simulink model "ASM_Traffic_MultiCore"  (R2026a)
settings: Solver=ode1  StartTime=SIM.tstart.v  StopTime=SIM.tend.v  FixedStep=SIM.StepSize.v
PostLoadFcn:
  | if any(exist('dsrtsu_mdlpostloadfcn', 'file') ~= 0), dsrtsu_mdlpostloadfcn('Execute', bdroot); end
  | try, asm_mdl_postloadfcn(bdroot, 'UpdateModel', 3600); catch, disp(lasterr); end,
InitFcn:
  | , if any(exist('rtifpga_mdlclblib', 'file') ~= 0), rtifpga_mdlclblib('Init', bdroot); end,
  | , if any(exist('dsmpb_private', 'file') ~= 0), dsmpb_private('dsmpb_mdlclblib', 'Init', bdroot); end,
model workspace (MAT data in the model file):
  asmReferencePath = [0 0.01 0.02 0.03 0.04 0.05 0.06 0.07 0.08 0.09 0.1 0.11 ... (350007 elements, 50001x7)]
  roadBounds : Simulink.Parameter (value not decoded)
  safetyAxes : Simulink.Parameter (value not decoded)
undefined symbols (not defined in the file): _to_, a0b2, ASM_BrakeHydraulics_DemoSystems, ASM_VehicleDynamics_DemoSystems, b98103fe8ad365046cd0, BrakeCircuit, controllerConfig, CPT, Crankshaft, DiscIntNeverNeededParam, dsmsi, FinalDriveAssembly, MDL, ModeSignals, mu, Pos_BrakePedal_Maneuver, rad, RefSignals, roadFamilyData, roadFamilyId, s_to_rpm, SIM, SoftECU, Suspension, Tire, Transmission
libraries: ASM_Traffic_lib x135, simulink x98, ASM_Utils_lib x77, ASM_VehicleDynamics_lib x70, ASM_Environment_lib x22, dsmpblib x20, dsmsilib x15, MDLD_Utils_lib x10, ASM_BrakeHydraulics_lib x3, sl_discontinuities x2
(part 7 of 65)

== system ASM_Traffic_MultiCore/AnimationInterface/ANIMATION_INTERFACE/ASM_Vehicle_Instruments ==
  VehicleDynamics_Animation : Inport
  Environment_Animation : Inport  Port=2
  Drivetrain_Animation : Inport  Port=3
  Bus Selector1 : BusSelector  OutputSignals=v_x_Vehicle_CoG[km|h],a_y_Vehicle_CoG[m|s2],YawRate_Vehicle_CoG[deg|s]
  Bus Selector15 : BusSelector  OutputSignals=n_Engine[rpm],Gear[]
  Bus Selector2 : BusSelector  OutputSignals=s_Vehicle[m],Angle_Yaw_Vehicle_CoorSys_E[deg]
  Bus Selector4 : BusSelector  OutputSignals=s_Veh_Road[m],ManeuverTime[s],ManeuverState[]
  Enable_Data_Transfer : Constant
  Vehicle_Instruments : dsmsilib/dsmsi_simulation_data_objects_BL1  Priority=10001  parameterStr="{\"Version\":1,\"TransformInput\":false,\"EnableInput\":true,\"Objects\":[{\"Oid\":1,\"Name\":\"Speed\",\"TypeClass\":{\"Name\":\"Signal\",\"Class\":3,\"SignalProperty\":{\"InstrumentInput\":\"Input port\",\"Description\":null,\"Unit\":\"km/h\",\"Type\":0,\"Length\":1,\"ObjectsCount\":1},\"TransformationProperty\":null,\"PositionAndScaleProperty\":null,\"PositionProperty\":null},\"Children\":[]},{\"Oid\":2,\"Name\":\"LatAcc\",\"TypeClass\":{\"Name\":\"Signal\",\"Class\":3,\"SignalProperty\":{\"InstrumentInput\":\"Input port\",\"Description\":null,\"Unit\":\"m/s2\",\"Type\":0,\"Length\":1,\"ObjectsCount\":1},\"TransformationProperty\":null,\"PositionAndScaleProperty\":null,\"PositionProperty\":null},\"Children\":[]},{\"Oid\":3,\"Name\":\"YawRate\",\"TypeClass\":{\"Name\":\"Signal\",\"Class\":3,\"SignalProperty\":{\"InstrumentInput\":\"Input port\",\"Description\":null,\"Unit\":\"deg/s\",\"Type\":0,\"Length\":1,\"ObjectsCount\":1},\"TransformationProperty\":null,\"PositionAndScaleProperty\":null,\"PositionProperty\":null},\"Children\":[]},{\"Oid\":4,\"Name\":\"Engine\",\"TypeClass\":{\"Name\":\"Signal\",\"Class\":3,\"SignalProperty\":{\"InstrumentInput\":\"Input port\",\"Description\":null,\"Unit\":\"rpm\",\"Type\":0,\"Length\":1,\"ObjectsCount\":1},\"TransformationProperty\":null,\"PositionAndScaleProperty\":null,\"PositionProperty\":null},\"Children\":[]},{\"Oid\":5,\"Name\":\"Gear\",\"TypeClass\":{\"Name\":\"Signal\",\"Class\":3,\"SignalProperty\":{\"InstrumentInput\":\"Input port\",\"Description\":null,\"Unit\":null,\"Type\":0,\"Length\":1,\"ObjectsCount\":1},\"TransformationProperty\":null,\"PositionAndScaleProperty\":null,\"PositionProperty\":null},\"Children\":[]},{\"Oid\":6,\"Name\":\"s_Road\",\"TypeClass\":{\"Name\":\"Signal\",\"Class\":3,\"SignalProperty\":{\"InstrumentInput\":\"Input port\",\"Description\":null,\"Unit\":\"m\",\"Type\":0,\"Length\":1,\"ObjectsCount\":1},\"TransformationProperty\":null,\"PositionAndScaleProperty\":null,\"PositionProperty\":null},\"Children\":[]},{\"Oid\":7,\"Name\":\"ManeuverTime\",\"TypeClass\":{\"Name\":\"Signal\",\"Class\":3,\"SignalProperty\":{\"InstrumentInput\":\"Input port\",\"Description\":null,\"Unit\":\"s\",\"Type\":0,\"Length\":1,\"ObjectsCount\":1},\"TransformationProperty\":null,\"PositionAndScaleProperty\":null,\"PositionProperty\":null},\"Children\":[]},{\"Oid\":8,\"Name\":\"ManeuverState\",\"TypeClass\":{\"Name\":\"Signal\",\"Class\":3,\"SignalProperty\":{\"InstrumentInput\":\"Input port\",\"Description\":null,\"Unit\":null,\"Type\":0,\"Length\":1,\"ObjectsCount\":1},\"TransformationProperty\":null,\"PositionAndScaleProperty\":null,\"PositionProperty\":null},\"Children\":[]},{\"Oid\":9,\"Name\":\"DrivenDistance\",\"TypeClass\":{\"Name\":\"Signal\",\"Class\":3,\"SignalProperty\":{\"InstrumentInput\":\"Input port\",\"Description\":null,\"Unit\":\"m\",\"Type\":0,\"Length\":1,\"ObjectsCount\":1},\"TransformationProperty\":null,\"PositionAndScaleProperty\":null,\"PositionProperty\":null},\"Children\":[]},{\"Oid\":10,\"Name\":\"YawAngle\",\"TypeClass\":{\"Name\":\"Signal\",\"Class\":3,\"SignalProperty\":{\"InstrumentInput\":\"Input port\",\"Description\":null,\"Unit\":\"deg\",\"Type\":0,\"Length\":1,\"ObjectsCount\":1},\"TransformationProperty\":null,\"PositionAndScaleProperty\":null,\"PositionProperty\":null},\"Children\":[]}]}"  evalStr=dsmsi(gcb, 'EvalJson')  sampleTime=-1  globalBlockId=0  objectsBlockId=dsmsi(gcb, 'GetObjectBlockId')  objectsBlockGuiOpen=dsmsi(gcb, 'GetSdoGuiStatus')  dialogIsOpen=0  blockVersion=60  highPrecision=0  validNameBckp=Vehicle_Instruments
      settings: SourceProductName=dSPACE MSI Blockset
  wires:
  Enable_Data_Transfer/1 -> Vehicle_Instruments/1
  Environment_Animation/1 -> Bus Selector4/1
  Bus Selector2/2 -> Vehicle_Instruments/11  "<Angle_Yaw_Vehicle_CoorSys_E[deg]>"
  Bus Selector2/1 -> Vehicle_Instruments/10  "<s_Vehicle[m]>"
  Bus Selector4/1 -> Vehicle_Instruments/7  "<s_Veh_Road[m]>"
  Bus Selector4/2 -> Vehicle_Instruments/8  "<ManeuverTime[s]>"
  Bus Selector1/2 -> Vehicle_Instruments/3  "<a_y_Vehicle_CoG[m|s2]>"
  Bus Selector1/1 -> Vehicle_Instruments/2  "<v_x_Vehicle_CoG[km|h]>"
  Bus Selector1/3 -> Vehicle_Instruments/4  "<YawRate_Vehicle_CoG[deg|s]>"
  Bus Selector4/3 -> Vehicle_Instruments/9  "<ManeuverState[]>"
  VehicleDynamics_Animation/1 -> Bus Selector1/1, Bus Selector2/1
  Drivetrain_Animation/1 -> Bus Selector15/1
  Bus Selector15/1 -> Vehicle_Instruments/5  "<n_Engine[rpm]>"
  Bus Selector15/2 -> Vehicle_Instruments/6  "<Gear[]>"

== system ASM_Traffic_MultiCore/AnimationInterface/ANIMATION_INTERFACE/ASM_Vehicle_Occupants ==
  Environment_Animation : Inport
  Bus Selector : BusSelector  OutputSignals=UserSignals_Customized.DriverMonitoring.DriverGazeLocation[],UserSignals_Customized.DriverMonitoring.DriverAnimation[],UserSignals_Customized.DriverMonitoring.DriverLizardOwlRatio[]
  Enable_Data_Transfer : Constant
  Vehicle_Occupants : dsmsilib/dsmsi_simulation_data_objects_BL1  Priority=10001  parameterStr="{\"Version\":1,\"TransformInput\":false,\"EnableInput\":true,\"Objects\":[{\"Oid\":1,\"Name\":\"Driver\",\"TypeClass\":{\"Name\":\"Transformation\",\"Class\":1,\"SignalProperty\":null,\"TransformationProperty\":{\"ObjectsCount\":1,\"TransformMatrixIn\":false,\"TransformMatrixOut\":false,\"AngleInterpretation\":0,\"TransformationOrder\":0,\"RotationOrder\":0,\"TranslationAsParameter\":true,\"Translation\":\"[0 0 0]\",\"RotationAsParameter\":true,\"Rotation\":\"[0 0 0]\",\"ScalingAsParameter\":true,\"Scaling\":\"[1 1 1]\"},\"PositionAndScaleProperty\":null,\"PositionProperty\":null},\"Children\":[{\"Oid\":2,\"Name\":\"DMS_GazeLocation\",\"TypeClass\":{\"Name\":\"Signal\",\"Class\":3,\"SignalProperty\":{\"ObjectsCount\":1,\"InstrumentInput\":\"Input port\",\"Description\":null,\"Unit\":null,\"Type\":0,\"Length\":1},\"TransformationProperty\":null,\"PositionAndScaleProperty\":null,\"PositionProperty\":null},\"Children\":[]},{\"Oid\":3,\"Name\":\"DMS_DriverAnimation\",\"TypeClass\":{\"Name\":\"Signal\",\"Class\":3,\"SignalProperty\":{\"ObjectsCount\":1,\"InstrumentInput\":\"Input port\",\"Description\":null,\"Unit\":null,\"Type\":0,\"Length\":1},\"TransformationProperty\":null,\"PositionAndScaleProperty\":null,\"PositionProperty\":null},\"Children\":[]},{\"Oid\":4,\"Name\":\"DMS_LizardOwlRatio\",\"TypeClass\":{\"Name\":\"Signal\",\"Class\":3,\"SignalProperty\":{\"ObjectsCount\":1,\"InstrumentInput\":\"Input port\",\"Description\":null,\"Unit\":null,\"Type\":0,\"Length\":1},\"TransformationProperty\":null,\"PositionAndScaleProperty\":null,\"PositionProperty\":null},\"Children\":[]}]}]}"  evalStr=dsmsi(gcb, 'EvalJson')  sampleTime=-1  globalBlockId=0  objectsBlockId=dsmsi(gcb, 'GetObjectBlockId')  objectsBlockGuiOpen=dsmsi(gcb, 'GetSdoGuiStatus')  dialogIsOpen=0  blockVersion=60  highPrecision=0  validNameBckp=Vehicle_Occupants
      settings: SourceProductName=dSPACE MSI Blockset
  wires:
  Bus Selector/3 -> Vehicle_Occupants/4  "<DriverLizardOwlRatio[]>"
  Bus Selector/2 -> Vehicle_Occupants/3  "<DriverAnimation[]>"
  Bus Selector/1 -> Vehicle_Occupants/2  "<DriverGazeLocation[]>"
  Enable_Data_Transfer/1 -> Vehicle_Occupants/1
  Environment_Animation/1 -> Bus Selector/1

== system ASM_Traffic_MultiCore/AnimationInterface/ANIMATION_INTERFACE/Activate_Animation ==

== system ASM_Traffic_MultiCore/AnimationInterface/ANIMATION_INTERFACE/Activate_Animation1 ==

== system ASM_Traffic_MultiCore/AnimationInterface/ANIMATION_INTERFACE/Activate_Animation2 ==

== system ASM_Traffic_MultiCore/AnimationInterface/ANIMATION_INTERFACE/Activate_Animation3 ==

== system ASM_Traffic_MultiCore/AnimationInterface/ANIMATION_INTERFACE/Activate_Animation4 ==

== system ASM_Traffic_MultiCore/AnimationInterface/ANIMATION_INTERFACE/Activate_Animation5 ==

== system ASM_Traffic_MultiCore/AnimationInterface/ANIMATION_INTERFACE/Activate_Animation6 ==

== system ASM_Traffic_MultiCore/AnimationInterface/ANIMATION_INTERFACE/Bounding_Boxes ==
  Environment_Animation : Inport
  BoundingBox_1 : Subsystem
  BoundingBox_10 : Subsystem
  BoundingBox_2 : Subsystem
  BoundingBox_3 : Subsystem
  BoundingBox_4 : Subsystem
  BoundingBox_5 : Subsystem
  BoundingBox_6 : Subsystem
  BoundingBox_7 : Subsystem
  BoundingBox_8 : Subsystem
  BoundingBox_9 : Subsystem
  Bounding_Boxes : dsmsilib/dsmsi_simulation_data_objects_BL1  Priority=10001  parameterStr="{\"Version\":1,\"TransformInput\":false,\"EnableInput\":true,\"Objects\":[{\"Name\":\"Boundingbox_01\",\"TypeClass\":{\"Name\":\"Transformation\",\"Class\":1,\"SignalProperty\":null,\"TransformationProperty\":{\"TransformMatrixIn\":false,\"TransformMatrixOut\":false,\"AngleInterpretation\":0,\"TransformationOrder\":0,\"RotationOrder\":0,\"TranslationAsParameter\":false,\"Translation\":\"[0 0 0]\",\"RotationAsParameter\":false,\"Rotation\":\"[0 0 0]\",\"ScalingAsParameter\":false,\"Scaling\":\"[1 1 1]\",\"ObjectsCount\":1},\"PositionAndScaleProperty\":null,\"PositionProperty\":null},\"Children\":[],\"Oid\":1},{\"Name\":\"Boundingbox_02\",\"TypeClass\":{\"Name\":\"Transformation\",\"Class\":1,\"SignalProperty\":null,\"TransformationProperty\":{\"TransformMatrixIn\":false,\"TransformMatrixOut\":false,\"AngleInterpretation\":0,\"TransformationOrder\":0,\"RotationOrder\":0,\"TranslationAsParameter\":false,\"Translation\":\"[0 0 0]\",\"RotationAsParameter\":false,\"Rotation\":\"[0 0 0]\",\"ScalingAsParameter\":false,\"Scaling\":\"[1 1 1]\",\"ObjectsCount\":1},\"PositionAndScaleProperty\":null,\"PositionProperty\":null},\"Children\":[],\"Oid\":2},{\"Name\":\"Boundingbox_03\",\"TypeClass\":{\"Name\":\"Transformation\",\"Class\":1,\"SignalProperty\":null,\"TransformationProperty\":{\"TransformMatrixIn\":false,\"TransformMatrixOut\":false,\"AngleInterpretation\":0,\"TransformationOrder\":0,\"RotationOrder\":0,\"TranslationAsParameter\":false,\"Translation\":\"[0 0 0]\",\"RotationAsParameter\":false,\"Rotation\":\"[0 0 0]\",\"ScalingAsParameter\":false,\"Scaling\":\"[1 1 1]\",\"ObjectsCount\":1},\"PositionAndScaleProperty\":null,\"PositionProperty\":null},\"Children\":[],\"Oid\":3},{\"Name\":\"Boundingbox_04\",\"TypeClass\":{\"Name\":\"Transformation\",\"Class\":1,\"SignalProperty\":null,\"TransformationProperty\":{\"TransformMatrixIn\":false,\"TransformMatrixOut\":false,\"AngleInterpretation\":0,\"TransformationOrder\":0,\"RotationOrder\":0,\"TranslationAsParameter\":false,\"Translation\":\"[0 0 0]\",\"RotationAsParameter\":false,\"Rotation\":\"[0 0 0]\",\"ScalingAsParameter\":false,\"Scaling\":\"[1 1 1]\",\"ObjectsCount\":1},\"PositionAndScaleProperty\":null,\"PositionProperty\":null},\"Children\":[],\"Oid\":4},{\"Name\":\"Boundingbox_05\",\"TypeClass\":{\"Name\":\"Transformation\",\"Class\":1,\"SignalProperty\":null,\"TransformationProperty\":{\"TransformMatrixIn\":false,\"TransformMatrixOut\":false,\"AngleInterpretation\":0,\"TransformationOrder\":0,\"RotationOrder\":0,\"TranslationAsParameter\":false,\"Translation\":\"[0 0 0]\",\"RotationAsParameter\":false,\"Rotation\":\"[0 0 0]\",\"ScalingAsParameter\":false,\"Scaling\":\"[1 1 1]\",\"ObjectsCount\":1},\"PositionAndScaleProperty\":null,\"PositionProperty\":null},\"Children\":[],\"Oid\":5},{\"Name\":\"Boundingbox_06\",\"TypeClass\":{\"Name\":\"Transformation\",\"Class\":1,\"SignalProperty\":null,\"TransformationProperty\":{\"TransformMatrixIn\":false,\"TransformMatrixOut\":false,\"AngleInterpretation\":0,\"TransformationOrder\":0,\"RotationOrder\":0,\"TranslationAsParameter\":false,\"Translation\":\"[0 0 0]\",\"RotationAsParameter\":false,\"Rotation\":\"[0 0 0]\",\"ScalingAsParameter\":false,\"Scaling\":\"[1 1 1]\",\"ObjectsCount\":1},\"PositionAndScaleProperty\":null,\"PositionProperty\":null},\"Children\":[],\"Oid\":6},{\"Name\":\"Boundingbox_07\",\"TypeClass\":{\"Name\":\"Transformation\",\"Class\":1,\"SignalProperty\":null,\"TransformationProperty\":{\"TransformMatrixIn\":false,\"TransformMatrixOut\":false,\"AngleInterpretation\":0,\"TransformationOrder\":0,\"RotationOrder\":0,\"TranslationAsParameter\":false,\"Translation\":\"[0 0 0]\",\"RotationAsParameter\":false,\"Rotation\":\"[0 0 0]\",\"ScalingAsParameter\":false,\"Scaling\":\"[1 1 1]\",\"ObjectsCount\":1},\"PositionAndScaleProperty\":null,\"PositionProperty\":null},\"Children\":[],\"Oid\":7},{\"Name\":\"Boundingbox_08\",\"TypeClass\":{\"Name\":\"Transformation\",\"Class\":1,\"SignalProperty\":null,\"TransformationProperty\":{\"TransformMatrixIn\":false,\"TransformMatrixOut\":false,\"AngleInterpretation\":0,\"TransformationOrder\":0,\"RotationOrder\":0,\"TranslationAsParameter\":false,\"Translation\":\"[0 0 0]\",\"RotationAsParameter\":false,\"Rotation\":\"[0 0 0]\",\"ScalingAsParameter\":false,\"Scaling\":\"[1 1 1]\",\"ObjectsCount\":1},\"PositionAndScaleProperty\":null,\"PositionProperty\":null},\"Children\":[],\"Oid\":8},{\"Name\":\"Boundingbox_09\",\"TypeClass\":{\"Name\":\"Transformation\",\"Class\":1,\"SignalProperty\":null,\"TransformationProperty\":{\"TransformMatrixIn\":false,\"TransformMatrixOut\":false,\"AngleInterpretation\":0,\"TransformationOrder\":0,\"RotationOrder\":0,\"TranslationAsParameter\":false,\"Translation\":\"[0 0 0]\",\"RotationAsParameter\":false,\"Rotation\":\"[0 0 0]\",\"ScalingAsParameter\":false,\"Scaling\":\"[1 1 1]\",\"ObjectsCount\":1},\"PositionAndScaleProperty\":null,\"PositionProperty\":null},\"Children\":[],\"Oid\":9},{\"Name\":\"Boundingbox_10\",\"TypeClass\":{\"Name\":\"Transformation\",\"Class\":1,\"SignalProperty\":null,\"TransformationProperty\":{\"TransformMatrixIn\":false,\"TransformMatrixOut\":false,\"AngleInterpretation\":0,\"TransformationOrder\":0,\"RotationOrder\":0,\"TranslationAsParameter\":false,\"Translation\":\"[0 0 0]\",\"RotationAsParameter\":false,\"Rotation\":\"[0 0 0]\",\"ScalingAsParameter\":false,\"Scaling\":\"[1 1 1]\",\"ObjectsCount\":1},\"PositionAndScaleProperty\":null,\"PositionProperty\":null},\"Children\":[],\"Oid\":10}]}"  evalStr=dsmsi(gcb, 'EvalJson')  sampleTime=-1  globalBlockId=0  objectsBlockId=dsmsi(gcb, 'GetObjectBlockId')  objectsBlockGuiOpen=dsmsi(gcb, 'GetSdoGuiStatus')  dialogIsOpen=0  blockVersion=60  highPrecision=0  validNameBckp=Bounding_Boxes
      settings: SourceProductName=dSPACE MSI Blockset
  Constant : Constant
  Constant1 : Constant  Value=2
  Constant2 : Constant  Value=3
  Constant3 : Constant  Value=4
  Constant4 : Constant  Value=5
  Constant5 : Constant  Value=6
  Constant6 : Constant  Value=7
  Constant7 : Constant  Value=8
  Constant8 : Constant  Value=9
  Constant9 : Constant  Value=10
  EnableBoxVisualization : Subsystem
  Enable_Data_Transfer : Constant
  wires:
  Enable_Data_Transfer/1 -> Bounding_Boxes/1
  BoundingBox_9/1(Pos_CoorSysE[m]) -> Bounding_Boxes/26
  BoundingBox_9/2(Angle_CoorSysE[m]) -> Bounding_Boxes/27
  BoundingBox_9/3(Dimensions[m]) -> Bounding_Boxes/28
  BoundingBox_10/1(Pos_CoorSysE[m]) -> Bounding_Boxes/29
  BoundingBox_10/2(Angle_CoorSysE[m]) -> Bounding_Boxes/30
  BoundingBox_10/3(Dimensions[m]) -> Bounding_Boxes/31
  BoundingBox_5/1(Pos_CoorSysE[m]) -> Bounding_Boxes/14
  BoundingBox_5/2(Angle_CoorSysE[m]) -> Bounding_Boxes/15
  BoundingBox_5/3(Dimensions[m]) -> Bounding_Boxes/16
  BoundingBox_6/1(Pos_CoorSysE[m]) -> Bounding_Boxes/17
  BoundingBox_6/2(Angle_CoorSysE[m]) -> Bounding_Boxes/18
  BoundingBox_6/3(Dimensions[m]) -> Bounding_Boxes/19
  BoundingBox_8/3(Dimensions[m]) -> Bounding_Boxes/25
  BoundingBox_8/2(Angle_CoorSysE[m]) -> Bounding_Boxes/24
  BoundingBox_8/1(Pos_CoorSysE[m]) -> Bounding_Boxes/23
  BoundingBox_7/3(Dimensions[m]) -> Bounding_Boxes/22
  BoundingBox_7/2(Angle_CoorSysE[m]) -> Bounding_Boxes/21
  BoundingBox_7/1(Pos_CoorSysE[m]) -> Bounding_Boxes/20
  BoundingBox_3/1(Pos_CoorSysE[m]) -> Bounding_Boxes/8
  BoundingBox_3/2(Angle_CoorSysE[m]) -> Bounding_Boxes/9
  BoundingBox_3/3(Dimensions[m]) -> Bounding_Boxes/10
  BoundingBox_4/1(Pos_CoorSysE[m]) -> Bounding_Boxes/11
  BoundingBox_4/2(Angle_CoorSysE[m]) -> Bounding_Boxes/12
  BoundingBox_4/3(Dimensions[m]) -> Bounding_Boxes/13
  BoundingBox_2/3(Dimensions[m]) -> Bounding_Boxes/7
  BoundingBox_2/2(Angle_CoorSysE[m]) -> Bounding_Boxes/6
  BoundingBox_2/1(Pos_CoorSysE[m]) -> Bounding_Boxes/5
  EnableBoxVisualization/1(BoundigBoxes_Animation) -> BoundingBox_10/2(BoundigBoxes_Animation), BoundingBox_9/2(BoundigBoxes_Animation), BoundingBox_8/2(BoundigBoxes_Animation), BoundingBox_7/2(BoundigBoxes_Animation), BoundingBox_6/2(BoundigBoxes_Animation), BoundingBox_5/2(BoundigBoxes_Animation), BoundingBox_4/2(BoundigBoxes_Animation), BoundingBox_3/2(BoundigBoxes_Animation), BoundingBox_2/2(BoundigBoxes_Animation), BoundingBox_1/2(BoundigBoxes_Animation)
  Environment_Animation/1 -> EnableBoxVisualization/1(Environment_Animation)
  BoundingBox_1/3(Dimensions[m]) -> Bounding_Boxes/4
  BoundingBox_1/2(Angle_CoorSysE[m]) -> Bounding_Boxes/3
  BoundingBox_1/1(Pos_CoorSysE[m]) -> Bounding_Boxes/2
  Constant/1 -> BoundingBox_1/1(Index[])
  Constant1/1 -> BoundingBox_2/1(Index[])
  Constant2/1 -> BoundingBox_3/1(Index[])
  Constant3/1 -> BoundingBox_4/1(Index[])
  Constant4/1 -> BoundingBox_5/1(Index[])
  Constant5/1 -> BoundingBox_6/1(Index[])
  Constant6/1 -> BoundingBox_7/1(Index[])
  Constant7/1 -> BoundingBox_8/1(Index[])
  Constant8/1 -> BoundingBox_9/1(Index[])
  Constant9/1 -> BoundingBox_10/1(Index[])

== system ASM_Traffic_MultiCore/AnimationInterface/ANIMATION_INTERFACE/Connection_Settings ==
  Environment_Animation : Inport
  Communication_Service : Subsystem  Tag=AnimationInterface_SIL
  Communication_Service_Common_Signals : Subsystem
  Display1 : Display
      settings: Format=decimal (Stored Integer)
  Ethernet_TCP : Subsystem  Tag=AnimationInterface_SIL  Commented=on
  MultiportSwitch{,1..3} (4 alike) : MultiPortSwitch  DataPortOrder=Zero-based contiguous  Inputs=2  zeroidx=on  SaturateOnIntegerOverflow=off  InputSameDT=off
  Sw_CommunicationMethod[0TCP|1ComService] : Constant
  dsmsi_connection_settings_BL1 : dsmsilib/dsmsi_connection_settings_BL1  Priority=10009  rateDividerPort=off  rateDivider=1  application=MotionDesk  reuse=off  source=dsmsilib/dsmsi_connection_settings_BL1  sendObjects=on  comment=Observer  txBufferSize=65507  enableTxBufferSize=off  globalBlockId=dsmsi(gcb, 'GetId')  sourceId=0  numberOfObjectBlocks=dsmsi(gcb, 'CountObjectBlocks')  numberOfGlobalBlocks=dsmsi(gcb, 'CountGlobalBlocks')  numberOfSensorFailureBlocks=dsmsi(gcb, 'CountSensorFailureBlocks')  uuid=7fbc0f5c-1ab5-4f7c-8d42-b98103fe8ad365046cd0-299c-42cd-a0b2-8824978edec42fda6c2b-1778-4453-86b3-4d675bee6ea0  countPipelines=dsmsi(gcb, 'CountPipelines')  debugCom=off  forceInitData=0  blockVersion=60  dialogIsOpen='0'  validNameBckp=dsmsi_connection_settings_BL1  updateFlag=0  Tx_rate_n=1  txRate=1  txRateInputPort=off
      settings: AttributesFormatString=%<comment>  SourceProductName=dSPACE MSI Blockset
  wires:
  Communication_Service_Common_Signals/2(Reset[0|1]) -> Communication_Service/4(Reset[0|1])
  Communication_Service_Common_Signals/1(ReferenceTime[s]) -> Communication_Service/3(ReferenceTime[s])
  Environment_Animation/1 -> Communication_Service_Common_Signals/1(Environment_Animation)
  dsmsi_connection_settings_BL1/1 -> Display1/1
  dsmsi_connection_settings_BL1/2 -> Ethernet_TCP/1(Tx_Length), Communication_Service/1(Tx_Length)
  dsmsi_connection_settings_BL1/3 -> Ethernet_TCP/2(Tx_Data), Communication_Service/2(Tx_Data)
  Communication_Service/1(Connected) -> MultiportSwitch/3
  Communication_Service/2(Tx_Sent_bytes) -> MultiportSwitch1/3
  Communication_Service/3(Rx_Length) -> MultiportSwitch2/3
  Communication_Service/4(Rx_Data) -> MultiportSwitch3/3
  Sw_CommunicationMethod[0TCP|1ComService]/1 -> MultiportSwitch/1, MultiportSwitch1/1, MultiportSwitch2/1, MultiportSwitch3/1
  MultiportSwitch/1 -> dsmsi_connection_settings_BL1/1
  MultiportSwitch1/1 -> dsmsi_connection_settings_BL1/2
  MultiportSwitch2/1 -> dsmsi_connection_settings_BL1/3
  MultiportSwitch3/1 -> dsmsi_connection_settings_BL1/4
  Ethernet_TCP/1(Connected) -> MultiportSwitch/2
  Ethernet_TCP/2(Tx_Sent_bytes) -> MultiportSwitch1/2
  Ethernet_TCP/3(Rx_Length) -> MultiportSwitch2/2
  Ethernet_TCP/4(Rx_Data) -> MultiportSwitch3/2

== system ASM_Traffic_MultiCore/AnimationInterface/ANIMATION_INTERFACE/Data_Streams_Instruments ==
  Environment_Animation : Inport
  Bus Selector2 : BusSelector  OutputSignals=Objects_DataStreams[].DataStream_1[].DataStream_1[],Objects_DataStreams[].DataStream_2[].DataStream_2[],Objects_DataStreams[].DataStream_3[].DataStream_3[],Objects_DataStreams[].DataStream_4[].DataStream_4[],Objects_DataStreams[].DataStream_5[].DataStream_5[],Objects_DataStreams[].DataStream_6[].DataStream_6[],Objects_DataStreams[].DataStream_7[].DataStream_7[],Objects_DataStreams[].DataStream_8[].DataStream_8[]
  Enable_Data_Transfer : Constant
  Objects_DataStreams_Instruments : dsmsilib/dsmsi_simulation_data_objects_BL1  Priority=10001  parameterStr="{\"Version\":1,\"TransformInput\":false,\"EnableInput\":true,\"Objects\":[{\"Name\":\"Obj_DataStream_001\",\"TypeClass\":{\"Name\":\"Signal\",\"Class\":3,\"SignalProperty\":{\"Description\":null,\"Unit\":null,\"Type\":0,\"Length\":1,\"ObjectsCount\":1},\"TransformationProperty\":null,\"PositionAndScaleProperty\":null,\"PositionProperty\":null},\"Children\":[],\"Oid\":1},{\"Name\":\"Obj_DataStream_002\",\"TypeClass\":{\"Name\":\"Signal\",\"Class\":3,\"SignalProperty\":{\"Description\":null,\"Unit\":null,\"Type\":0,\"Length\":1,\"ObjectsCount\":1},\"TransformationProperty\":null,\"PositionAndScaleProperty\":null,\"PositionProperty\":null},\"Children\":[],\"Oid\":2},{\"Name\":\"Obj_DataStream_003\",\"TypeClass\":{\"Name\":\"Signal\",\"Class\":3,\"SignalProperty\":{\"Description\":null,\"Unit\":null,\"Type\":0,\"Length\":1,\"ObjectsCount\":1},\"TransformationProperty\":null,\"PositionAndScaleProperty\":null,\"PositionProperty\":null},\"Children\":[],\"Oid\":3},{\"Name\":\"Obj_DataStream_004\",\"TypeClass\":{\"Name\":\"Signal\",\"Class\":3,\"SignalProperty\":{\"Description\":null,\"Unit\":null,\"Type\":0,\"Length\":1,\"ObjectsCount\":1},\"TransformationProperty\":null,\"PositionAndScaleProperty\":null,\"PositionProperty\":null},\"Children\":[],\"Oid\":4},{\"Name\":\"Obj_DataStream_005\",\"TypeClass\":{\"Name\":\"Signal\",\"Class\":3,\"SignalProperty\":{\"Description\":null,\"Unit\":null,\"Type\":0,\"Length\":1,\"ObjectsCount\":1},\"TransformationProperty\":null,\"PositionAndScaleProperty\":null,\"PositionProperty\":null},\"Children\":[],\"Oid\":5},{\"Name\":\"Obj_DataStream_006\",\"TypeClass\":{\"Name\":\"Signal\",\"Class\":3,\"SignalProperty\":{\"Description\":null,\"Unit\":null,\"Type\":0,\"Length\":1,\"ObjectsCount\":1},\"TransformationProperty\":null,\"PositionAndScaleProperty\":null,\"PositionProperty\":null},\"Children\":[],\"Oid\":6},{\"Name\":\"Obj_DataStream_007\",\"TypeClass\":{\"Name\":\"Signal\",\"Class\":3,\"SignalProperty\":{\"Description\":null,\"Unit\":null,\"Type\":0,\"Length\":1,\"ObjectsCount\":1},\"TransformationProperty\":null,\"PositionAndScaleProperty\":null,\"PositionProperty\":null},\"Children\":[],\"Oid\":7},{\"Name\":\"Obj_DataStream_008\",\"TypeClass\":{\"Name\":\"Signal\",\"Class\":3,\"SignalProperty\":{\"Description\":null,\"Unit\":null,\"Type\":0,\"Length\":1,\"ObjectsCount\":1},\"TransformationProperty\":null,\"PositionAndScaleProperty\":null,\"PositionProperty\":null},\"Children\":[],\"Oid\":8}]}"  evalStr=dsmsi(gcb, 'EvalJson')  sampleTime=-1  globalBlockId=0  objectsBlockId=dsmsi(gcb, 'GetObjectBlockId')  objectsBlockGuiOpen=dsmsi(gcb, 'GetSdoGuiStatus')  dialogIsOpen=0  blockVersion=60  highPrecision=0  validNameBckp=Objects_DataStreams_Instruments
      settings: SourceProductName=dSPACE MSI Blockset
  wires:
  Environment_Animation/1 -> Bus Selector2/1
  Enable_Data_Transfer/1 -> Objects_DataStreams_Instruments/1
  Bus Selector2/2 -> Objects_DataStreams_Instruments/3  "<DataStream_2[]>"
  Bus Selector2/7 -> Objects_DataStreams_Instruments/8  "<DataStream_7[]>"
  Bus Selector2/4 -> Objects_DataStreams_Instruments/5  "<DataStream_4[]>"
  Bus Selector2/6 -> Objects_DataStreams_Instruments/7  "<DataStream_6[]>"
  Bus Selector2/8 -> Objects_DataStreams_Instruments/9  "<DataStream_8[]>"
  Bus Selector2/1 -> Objects_DataStreams_Instruments/2  "<DataStream_1[]>"
  Bus Selector2/3 -> Objects_DataStreams_Instruments/4  "<DataStream_3[]>"
  Bus Selector2/5 -> Objects_DataStreams_Instruments/6  "<DataStream_5[]>"
